simulink library "Lib_Piccolo"  (R2018b)
settings: Solver=VariableStepAuto  StartTime=0.0  StopTime=10.0  RelTol=1e-3
values from neighbouring files (symbols this model uses):
  AccelErrInt2Brakes = 0.15    [SimulationControlConfig16P.m]    (also in SimulationControlConfig16P_LEGACY.m; SimulationControlConfigTAILLESS.m = 0.2; SimulationControlConfigUTAIL.m = 0.2)
  AileronMax = 25    [SimulationControlConfig16P.m]    (also in SimulationControlConfig16P_LEGACY.m; SimulationControlConfigTAILLESS.m; SimulationControlConfigUTAIL.m)
  AileronPower = 0.00268    [SimulationControlConfig16P.m]    (also in SimulationControlConfig16P_LEGACY.m; SimulationControlConfigTAILLESS.m; SimulationControlConfigUTAIL.m)
  AileronSurfaceMax = 45    [SimulationControlConfig16P.m]    (also in SimulationControlConfig16P_LEGACY.m)
  AileronTrim = 0    [SimulationControlConfig16P.m]    (also in SimulationControlConfig16P_LEGACY.m; SimulationControlConfigTAILLESS.m; SimulationControlConfigUTAIL.m)
  Alt = 1000 + TerrainHeight    [SimulationStateConfig.m]
  AltCruise_m = testPlans(testIndx).terrainElevation * 0.3048 + 200    [SimulationControlConfig16P.m]    (also in SimulationControlConfigTAILLESS.m = 1083; SimulationControlConfigUTAIL.m = testPlans(testIndx).terrainElevation * 0.3048 + 152)
  AltitudeRate2PitchCmdIntegratorInit = 0.1    [SimulationControlPre.m]
  AltMax = 10000    [SimulationControlConfig16P.m]    (also in SimulationControlConfig16P_LEGACY.m; SimulationControlConfigTAILLESS.m; SimulationControlConfigUTAIL.m)
  AltMaxAccel = 1.25    [SimulationControlConfig16P.m]    (also in SimulationControlConfig16P_LEGACY.m = 0.9; SimulationControlConfigTAILLESS.m = 1.7; SimulationControlConfigUTAIL.m = 2)
  AltMin = 0    [SimulationControlConfig16P.m]    (also in SimulationControlConfig16P_LEGACY.m; SimulationControlConfigTAILLESS.m; SimulationControlConfigUTAIL.m)
  AltRateCmd2Pitch = 0.50    (= 0.5)    [SimulationControlConfig16P.m]    (also in SimulationControlConfig16P_LEGACY.m = 0.6; SimulationControlConfigTAILLESS.m = 0.2; SimulationControlConfigUTAIL.m = 0.3)
  AltRateError2Pitch = 0.40    (= 0.4)    [SimulationControlConfig16P.m]    (also in SimulationControlConfig16P_LEGACY.m; SimulationControlConfigTAILLESS.m = 0.55; SimulationControlConfigUTAIL.m = 0.55)
  AltRateErrorInt2Pitch = 0.50    (= 0.5)    [SimulationControlConfig16P.m]    (also in SimulationControlConfig16P_LEGACY.m = 0.45; SimulationControlConfigTAILLESS.m; SimulationControlConfigUTAIL.m = 0.75)
  AltRateLpfCutOff = 3    [SimulationControlConfig16P.m]    (also in SimulationControlConfig16P_LEGACY.m; SimulationControlConfigTAILLESS.m = 2; SimulationControlConfigUTAIL.m = 2)
  AutoNosegear2Rudder = 26    [SimulationControlConfig16P.m]    (also in SimulationControlConfig16P_LEGACY.m; SimulationControlConfigTAILLESS.m = 25.2; SimulationControlConfigUTAIL.m = 14)
  b = 5.54    [SimulationControlConfig16P.m]    (also in SimulationControlConfig16P_LEGACY.m; SimulationControlConfigTAILLESS.m = 2.37; SimulationControlConfigUTAIL.m = 2.37)
  Bank2AileronIntegratorInit = 0    [SimulationControlPre.m]
  BankMax_User = BankMax_User/180*pi    (= 0.523598775598)    [SimulationControlConfig16P.m]    (also in SimulationControlConfig16P_LEGACY.m; SimulationControlConfigTAILLESS.m = 0.610865238198; SimulationControlConfigUTAIL.m = 0.628318530718)
  baseLegFlaps = 20    [SimulationControlConfig16P.m]    (also in SimulationControlConfig16P_LEGACY.m = 0; SimulationControlConfigTAILLESS.m = 15; SimulationControlConfigUTAIL.m = 10)
  C = GeneticOpt.C    [SimulationCostFunction.m]
  c = Sw/b    (= 0.841696750903)    [SimulationControlConfig16P.m]    (also in SimulationControlConfig16P_LEGACY.m; SimulationControlConfigTAILLESS.m = 0.354008438819; SimulationControlConfigUTAIL.m = 0.354008438819)
  cell2WheelFactorMG = 5.98    [SimulationSensorConfig16P_LEGACY.m]
  cell2WheelFactorNG = 1    [SimulationSensorConfig16P_LEGACY.m]
  cellSatMaxMG = 15000    [SimulationSensorConfig16P.m]    (also in SimulationSensorConfig16P_LEGACY.m; SimulationSensorConfigTAILLESS7P.m; SimulationSensorConfigUTAIL7P.m)
  cellSatMaxNG = 1000    [SimulationSensorConfig16P.m]    (also in SimulationSensorConfig16P_LEGACY.m; SimulationSensorConfigTAILLESS7P.m; SimulationSensorConfigUTAIL7P.m)
  cellSatMinMG = -15000    [SimulationSensorConfig16P.m]    (also in SimulationSensorConfig16P_LEGACY.m; SimulationSensorConfigTAILLESS7P.m; SimulationSensorConfigUTAIL7P.m)
  cellSatMinNG = -1000    [SimulationSensorConfig16P.m]    (also in SimulationSensorConfig16P_LEGACY.m; SimulationSensorConfigTAILLESS7P.m; SimulationSensorConfigUTAIL7P.m)
  CL_Limit = CL_Max    (= 0.54)    [SimulationControlConfig16P.m]    (also in SimulationControlConfig16P_LEGACY.m; SimulationControlConfigTAILLESS.m; SimulationControlConfigUTAIL.m = 0.53)
  CL_Max = 0.54    [SimulationControlConfig16P.m]    (also in SimulationControlConfig16P_LEGACY.m; SimulationControlConfigTAILLESS.m; SimulationControlConfigUTAIL.m = 0.53)
  CL_Max_Nom = 0.465    [SimulationControlConfig16P.m]    (also in SimulationControlConfig16P_LEGACY.m; SimulationControlConfigTAILLESS.m = 0.39; SimulationControlConfigUTAIL.m)
  CL_Min = 0    [SimulationControlConfig16P.m]    (also in SimulationControlConfig16P_LEGACY.m; SimulationControlConfigTAILLESS.m; SimulationControlConfigUTAIL.m)
  ClimbMaxFraction = 0.35    [SimulationControlConfig16P.m]    (also in SimulationControlConfig16P_LEGACY.m = 0.24; SimulationControlConfigTAILLESS.m = 0.19; SimulationControlConfigUTAIL.m = 0.21)
  ClimboutMaxBank = 7.0    (= 7)    [SimulationControlConfig16P.m]    (also in SimulationControlConfig16P_LEGACY.m; SimulationControlConfigTAILLESS.m = 5; SimulationControlConfigUTAIL.m)
  ClimboutTimer = 7.0    (= 7)    [SimulationControlConfig16P.m]    (also in SimulationControlConfig16P_LEGACY.m; SimulationControlConfigTAILLESS.m; SimulationControlConfigUTAIL.m)
  dCl_per_dFlap = 0.005581818    [SimulationControlConfig16P.m]    (also in SimulationControlConfig16P_LEGACY.m = 0; SimulationControlConfigTAILLESS.m = 0; SimulationControlConfigUTAIL.m = 0)
  DecelerationCmd = 3.1    [SimulationControlConfig16P.m]    (also in SimulationControlConfig16P_LEGACY.m; SimulationControlConfigTAILLESS.m = 0.1; SimulationControlConfigUTAIL.m = 0.1)
  DeRotateLogicEndTimer = abs((NoseDownLimit_Deg-1)/DeRotateRamp_Dps)    [SimulationControlConfig16P.m]    (also in SimulationControlConfig16P_LEGACY.m; SimulationControlConfigTAILLESS.m; SimulationControlConfigUTAIL.m)
  DeRotateLogicHoldNoseUpTimer = 0.1    [SimulationControlConfig16P.m]    (also in SimulationControlConfig16P_LEGACY.m; SimulationControlConfigTAILLESS.m; SimulationControlConfigUTAIL.m)
  DeRotateLogicTimerTimeout = 2    [SimulationControlConfig16P.m]    (also in SimulationControlConfig16P_LEGACY.m; SimulationControlConfigTAILLESS.m; SimulationControlConfigUTAIL.m)
  DeRotateLowerCmdSaturation = 0    [SimulationControlConfig16P.m]    (also in SimulationControlConfig16P_LEGACY.m; SimulationControlConfigTAILLESS.m; SimulationControlConfigUTAIL.m)
  DeRotateRamp_Dps = 3    [SimulationControlConfig16P.m]    (also in SimulationControlConfig16P_LEGACY.m; SimulationControlConfigTAILLESS.m = 8; SimulationControlConfigUTAIL.m = 8)
  DeRotateUpperCmdSaturation = 7    [SimulationControlConfig16P.m]    (also in SimulationControlConfig16P_LEGACY.m; SimulationControlConfigTAILLESS.m; SimulationControlConfigUTAIL.m)
  DescentMaxFraction = 0.22    [SimulationControlConfig16P.m]    (also in SimulationControlConfig16P_LEGACY.m = 0.2; SimulationControlConfigTAILLESS.m = 0.17; SimulationControlConfigUTAIL.m = 0.17)
  DesktopSimTerrainOffset_m = 0.406    [SimulationAircraftConfig.m]
  downwindFlaps = 0    [SimulationControlConfig16P.m]    (also in SimulationControlConfig16P_LEGACY.m; SimulationControlConfigTAILLESS.m; SimulationControlConfigUTAIL.m)
  DP_init = 0.5*1.225*V_init^2    [SimulationControlConfig16P.m]    (also in SimulationControlConfig16P_LEGACY.m; SimulationControlConfigTAILLESS.m; SimulationControlConfigUTAIL.m)
  dscNoiseMG = 1    [SimulationSensorConfig16P_LEGACY.m]
  dscNoiseNG = 0.25    [SimulationSensorConfig16P_LEGACY.m]
  DSCnumBits = 24    [SimulationSensorConfig16P.m]    (also in SimulationSensorConfig16P_LEGACY.m; SimulationSensorConfigTAILLESS7P.m; SimulationSensorConfigUTAIL7P.m)
  DSCRangeMaxMG = 15000    [SimulationSensorConfig16P.m]    (also in SimulationSensorConfig16P_LEGACY.m; SimulationSensorConfigTAILLESS7P.m; SimulationSensorConfigUTAIL7P.m)
  DSCRangeMaxNG = 1000    [SimulationSensorConfig16P.m]    (also in SimulationSensorConfig16P_LEGACY.m; SimulationSensorConfigTAILLESS7P.m; SimulationSensorConfigUTAIL7P.m)
  DSCRangeMinMG = -15000    [SimulationSensorConfig16P.m]    (also in SimulationSensorConfig16P_LEGACY.m; SimulationSensorConfigTAILLESS7P.m; SimulationSensorConfigUTAIL7P.m)
  DSCRangeMinNG = -1000    [SimulationSensorConfig16P.m]    (also in SimulationSensorConfig16P_LEGACY.m; SimulationSensorConfigTAILLESS7P.m; SimulationSensorConfigUTAIL7P.m)
  dt = DLLSim.dt    [SimulationTimeStep.m]    (also in SimulationTrim.m = 0.02)
  EarlyTouchdownThreshold = 3.0    (= 3)    [SimulationControlConfig16P.m]    (also in SimulationControlConfig16P_LEGACY.m; SimulationControlConfigTAILLESS.m = 2.2; SimulationControlConfigUTAIL.m = 2.5)
  ElevatorDeflectionRate = 15    [SimulationControlConfig16P.m]    (also in SimulationControlConfig16P_LEGACY.m = 12; SimulationControlConfigTAILLESS.m = 10; SimulationControlConfigUTAIL.m = 12)
  ElevatorMax = 25    [SimulationControlConfig16P.m]    (also in SimulationControlConfig16P_LEGACY.m; SimulationControlConfigTAILLESS.m; SimulationControlConfigUTAIL.m)
  ElevatorPower = -0.002209    [SimulationControlConfig16P.m]    (also in SimulationControlConfig16P_LEGACY.m; SimulationControlConfigTAILLESS.m = -0.002956; SimulationControlConfigUTAIL.m = -0.00205983)
  ElevatorTrim = -3.5    [SimulationControlConfig16P.m]    (also in SimulationControlConfig16P_LEGACY.m; SimulationControlConfigTAILLESS.m = -6; SimulationControlConfigUTAIL.m = -8)
  elevonBias = 0    [SimulationControlConfig16P.m]    (also in SimulationControlConfig16P_LEGACY.m; SimulationControlConfigTAILLESS.m; SimulationControlConfigUTAIL.m)
  Enable_TAS_Protection = 0    [SimulationControlConfig16P.m]    (also in SimulationControlConfig16P_LEGACY.m; SimulationControlConfigTAILLESS.m; SimulationControlConfigUTAIL.m)
  EnableCrossTrackAbort = 1    [SimulationControlConfig16P.m]    (also in SimulationControlConfigTAILLESS.m; SimulationControlConfigUTAIL.m)
  EnergyBandwidth = 0.02    [SimulationControlConfig16P.m]    (also in SimulationControlConfig16P_LEGACY.m; SimulationControlConfigTAILLESS.m = 0.06; SimulationControlConfigUTAIL.m = 0.06)
  EngineLhFuelCut = 0    [SimulationAircraftConfig.m]
  EngineRhFuelCut = 0    [SimulationAircraftConfig.m]
  FastThrottleRate = 0.075    [SimulationControlConfig16P.m]    (also in SimulationControlConfig16P_LEGACY.m = 0.05; SimulationControlConfigTAILLESS.m = 0.1; SimulationControlConfigUTAIL.m = 0.1)
  FilterWarmUpTime = 2    [SimulationSensorConfig16P.m]    (also in SimulationSensorConfig16P_LEGACY.m; SimulationSensorConfigTAILLESS7P.m; SimulationSensorConfigUTAIL7P.m)
  finalApproachFlaps = 20    [SimulationControlConfig16P.m]    (also in SimulationControlConfig16P_LEGACY.m = 0; SimulationControlConfigTAILLESS.m = 22; SimulationControlConfigUTAIL.m = 10)
  FinalDescentSlope_Deg = testPlans(testIndx).descentSlope    [SimulationControlConfig16P.m]    (also in SimulationControlConfig16P_LEGACY.m; SimulationControlConfigTAILLESS.m; SimulationControlConfigUTAIL.m)
  flapMax = 0    [SimulationControlConfig16P.m]    (also in SimulationControlConfig16P_LEGACY.m; SimulationControlConfigTAILLESS.m; SimulationControlConfigUTAIL.m)
  flapRate = 7.5    [SimulationControlConfig16P.m]    (also in SimulationControlConfig16P_LEGACY.m; SimulationControlConfigTAILLESS.m = 6.6; SimulationControlConfigUTAIL.m)
  FlareHeight = 5    [SimulationControlConfig16P.m]    (also in SimulationControlConfig16P_LEGACY.m = 4.8; SimulationControlConfigTAILLESS.m = 2.5; SimulationControlConfigUTAIL.m = 2)
  FlareVerticalRate_mps = -0.4    [SimulationControlConfig16P.m]    (also in SimulationControlConfig16P_LEGACY.m = -0.5; SimulationControlConfigTAILLESS.m = -0.15; SimulationControlConfigUTAIL.m = -0.15)
  Fp_Aileron = 0.55*2*pi*RollRateLpfCutoff*dt    [SimulationControlConfig16P.m]    (also in SimulationControlConfig16P_LEGACY.m; SimulationControlConfigTAILLESS.m; SimulationControlConfigUTAIL.m)
  Fp_Alt = 0.55*AltBandwidth    (= 0.099)    [SimulationControlConfig16P.m]    (also in SimulationControlConfig16P_LEGACY.m; SimulationControlConfigTAILLESS.m = 0.587477826221; SimulationControlConfigUTAIL.m = 0.69115038379)
  Fp_AltRate = 0.55*2*pi*AltRateLpfCutOff*dt    [SimulationControlConfig16P.m]    (also in SimulationControlConfig16P_LEGACY.m; SimulationControlConfigTAILLESS.m; SimulationControlConfigUTAIL.m)
  Fp_Elevator = 0.55*2*pi*PitchRateLpfCutoff*dt    [SimulationControlConfig16P.m]    (also in SimulationControlConfig16P_LEGACY.m; SimulationControlConfigTAILLESS.m; SimulationControlConfigUTAIL.m)
  Fp_Energy = 0.55*2*pi*EnergyBandwidth    (= 0.069115038379)    [SimulationControlConfig16P.m]    (also in SimulationControlConfig16P_LEGACY.m; SimulationControlConfigTAILLESS.m = 0.207345115137; SimulationControlConfigUTAIL.m = 0.207345115137)
  Fp_Energy2 = 0.55*2*pi*EnergyBandwidth*dt    [SimulationControlConfig16P.m]    (also in SimulationControlConfig16P_LEGACY.m; SimulationControlConfigTAILLESS.m; SimulationControlConfigUTAIL.m)
  Fp_Pitch = 0.55*2*pi*PitchBandwidth    (= 2.76460153516)    [SimulationControlConfig16P.m]    (also in SimulationControlConfig16P_LEGACY.m = 3.11017672705; SimulationControlConfigTAILLESS.m = 3.80132711084; SimulationControlConfigUTAIL.m = 2.41902634326)
  Fp_Pitch_2 = 0.55*2*pi*PitchBandwidth*dt    [SimulationControlConfig16P.m]    (also in SimulationControlConfig16P_LEGACY.m; SimulationControlConfigTAILLESS.m; SimulationControlConfigUTAIL.m)
  Fp_Roll = RollBandwidth^2    (= 1)    [SimulationControlConfig16P.m]    (also in SimulationControlConfig16P_LEGACY.m = 1.44; SimulationControlConfigTAILLESS.m; SimulationControlConfigUTAIL.m)
  Fp_Rudder = 0.55*2*pi*YawRateLpfCutoff*dt    [SimulationControlConfig16P.m]    (also in SimulationControlConfig16P_LEGACY.m; SimulationControlConfigTAILLESS.m; SimulationControlConfigUTAIL.m)
  Fp_TAS = 0.55*2*pi*TASBandwidth    (= 0.103672557568)    [SimulationControlConfig16P.m]    (also in SimulationControlConfig16P_LEGACY.m; SimulationControlConfigTAILLESS.m = 0.172787595947; SimulationControlConfigUTAIL.m = 0.172787595947)
  Fp_TAS_Filter = 2*pi*TasLpfCutoff*dt    [SimulationControlConfig16P.m]    (also in SimulationControlConfig16P_LEGACY.m; SimulationControlConfigTAILLESS.m; SimulationControlConfigUTAIL.m)
  Fp_Turn = 0.55*2*pi*TurnErrLPFcutoff    (= 0.0345575191895)    [SimulationControlConfig16P.m]    (also in SimulationControlConfig16P_LEGACY.m; SimulationControlConfigTAILLESS.m = 0.172787595947; SimulationControlConfigUTAIL.m = 0.172787595947)
  Fp_TurnDerr = 0.55*2*pi*TurnDerivativeLPFcutoff    (= 0.0345575191895)    [SimulationControlConfig16P.m]    (also in SimulationControlConfig16P_LEGACY.m; SimulationControlConfigTAILLESS.m = 0.172787595947; SimulationControlConfigUTAIL.m = 0.172787595947)
  FTV = 3    [SimulationAircraftConfig.m]
  ftvStaticPositionError = 1/1.18    (= 0.847457627119)    [SimulationSensorConfig16P.m]    (also in SimulationSensorConfig16P_LEGACY.m; SimulationSensorConfigTAILLESS7P.m = 1; SimulationSensorConfigUTAIL7P.m = 1)
  g = 9.81    [SimulationStateConfig.m]
  GustSpd_Kts = testPlans(testIndx).gustSpd    [SimulationStateConfig.m]
  GustTriggerVal = testPlans(testIndx).gustTriggerVal    [SimulationStateConfig.m]
  HeadingErr2TurnRate = 0.5    [SimulationControlConfig16P.m]    (also in SimulationControlConfig16P_LEGACY.m; SimulationControlConfigTAILLESS.m; SimulationControlConfigUTAIL.m)
  HeadingErrDer2TurnRate = 0.3    [SimulationControlConfig16P.m]    (also in SimulationControlConfig16P_LEGACY.m; SimulationControlConfigTAILLESS.m; SimulationControlConfigUTAIL.m)
  IASbounce = IASstall*0.8    [SimulationControlPre.m]
  IAScruiseCMD = sqrt(2*m*9.81/(1.225*Sw*CL_cruise))    [SimulationControlConfig16P.m]    (also in SimulationControlConfig16P_LEGACY.m; SimulationControlConfigTAILLESS.m; SimulationControlConfigUTAIL.m)
  IASfinalCMD = 1.12 * IASmin    [SimulationControlConfig16P.m]    (also in SimulationControlConfig16P_LEGACY.m = 1.10 * IASmin; SimulationControlConfigTAILLESS.m = 1.10 * IASmin; SimulationControlConfigUTAIL.m = 1.15 * IASmin)
  IASflareCMD = IASstall    [SimulationControlConfig16P.m]    (also in SimulationControlConfig16P_LEGACY.m; SimulationControlConfigTAILLESS.m; SimulationControlConfigUTAIL.m)
  IASmax = 64    [SimulationControlConfig16P.m]    (also in SimulationControlConfig16P_LEGACY.m = 46; SimulationControlConfigTAILLESS.m = 38.58; SimulationControlConfigUTAIL.m = 35)
  IASmin = sqrt(2*m*9.81/(1.225*Sw*0.9*CL_Max_Nom))    [SimulationControlConfig16P.m]    (also in SimulationControlConfig16P_LEGACY.m; SimulationControlConfigTAILLESS.m; SimulationControlConfigUTAIL.m)
  IASshortCMD = IASstall    [SimulationControlConfig16P.m]    (also in SimulationControlConfig16P_LEGACY.m; SimulationControlConfigTAILLESS.m; SimulationControlConfigUTAIL.m)
  IASstall = sqrt(2*m*9.81/(1.225*Sw*CL_Max))    [SimulationControlConfig16P.m]    (also in SimulationControlConfig16P_LEGACY.m; SimulationControlConfigTAILLESS.m; SimulationControlConfigUTAIL.m)
  inFlight = 1    [SimulationControlConfig16P.m]    (also in SimulationControlConfigTAILLESS.m; SimulationControlConfigUTAIL.m)
  JetCatOffset = 5    [SimulationControlConfig16P.m]    (also in SimulationControlConfig16P_LEGACY.m)
  LaunchRollingElevator = -1.5    [SimulationControlConfig16P.m]    (also in SimulationControlConfig16P_LEGACY.m; SimulationControlConfigTAILLESS.m = 1; SimulationControlConfigUTAIL.m = 1)
  ldg_NosegearMax = 10    [SimulationControlConfig16P.m]    (also in SimulationControlConfig16P_LEGACY.m; SimulationControlConfigTAILLESS.m; SimulationControlConfigUTAIL.m)
  ldg_TrackVyErrInt2Nosegear = 0.1250    (= 0.125)    [SimulationControlConfig16P.m]    (also in SimulationControlConfig16P_LEGACY.m; SimulationControlConfigTAILLESS.m = 0.00714285714286; SimulationControlConfigUTAIL.m = 0.00714285714286)
  ldg_TrackVyErrPro2Nosegear = 0.35    [SimulationControlConfig16P.m]    (also in SimulationControlConfig16P_LEGACY.m; SimulationControlConfigTAILLESS.m = 0.0546666666667; SimulationControlConfigUTAIL.m = 0.0546666666667)
  ldg_TrackY2Vy = 0.07    [SimulationControlConfig16P.m]    (also in SimulationControlConfig16P_LEGACY.m; SimulationControlConfigTAILLESS.m = 0.17; SimulationControlConfigUTAIL.m = 0.17)
  ldg_Vy2NosegearScalingPower = 1.075    [SimulationControlConfig16P.m]    (also in SimulationControlConfig16P_LEGACY.m; SimulationControlConfigTAILLESS.m = 0.6; SimulationControlConfigUTAIL.m = 0.5)
  ldg_Y2VyScalingPower = 0.175    [SimulationControlConfig16P.m]    (also in SimulationControlConfig16P_LEGACY.m; SimulationControlConfigTAILLESS.m = 0; SimulationControlConfigUTAIL.m = 0)
  ldg_YawRate2Nosegear = 0.175    [SimulationControlConfig16P.m]    (also in SimulationControlConfig16P_LEGACY.m; SimulationControlConfigTAILLESS.m = 0.065; SimulationControlConfigUTAIL.m = 0.065)
  LiftSlope = 0.064285    [SimulationControlConfig16P.m]    (also in SimulationControlConfig16P_LEGACY.m; SimulationControlConfigTAILLESS.m = 0.058631; SimulationControlConfigUTAIL.m)
  LPFaileronInit = 0    [SimulationControlPre.m]
  LPFclestInit = 0    [SimulationControlPre.m]
  LPFenergyFFInit = 0    [SimulationControlPre.m]
  LPFtasInit = V_init + 2    [SimulationControlPre.m]
  LPFthrottleInit = ThrottleTrim    [SimulationControlPre.m]
  LPFturnErrInit = 0    [SimulationControlPre.m]
  ... (+115 more)
undefined symbols (not defined in the file or in its folder): abortFlag, alphaHPF, apmDelay, BRWNOUT, CRAWOR, CRAWUR, DiscIntNeverNeededParam, DLLSim, DLLSimStep, ECOMOR, ECOMUR, Fp_Tas, GustTrigger_HeightAgl_m, IPSTAT, LCINTEG, Ldg_Persist_Time, LOWER_FLAGS, MSG_ENABLE, NoiseStd, OLDVAL, OVERRIDE_ENABLE, OVERRIDE_VALUE, REBOOT, reversionEnable, revIASMax, revIASMin, revPitchMax, revPitchMin, revPitchRateMax, revRollMax, revRollRateMax, SAMPLE, SCALON, SensorModel, sigbuilder_block, Sim_Vx, Sim_Vy, Sim_Vz, Sim_Xpos, Sim_Ypos, Sim_Zpos, SYSOR, SYSUR, TARE, TEMPOR, TEMPUR, testIndx, testPlan, testPlans, Trim_piccoloInCmd, Trim_REFSI_FD_IN_nmodeCgShifterCmd_Ft, Trim_REFSI_FD_IN_nmodeFlapLhIBCmd_Deg, Trim_REFSI_FD_IN_nmodeFlapLhOBCmd_Deg, Trim_REFSI_FD_IN_nmodeFlapRhIBCmd_Deg, Trim_REFSI_FD_IN_nmodeFlapRhOBCmd_Deg, Trim_REFSI_FD_IN_nmodeSlatLhCmd_Deg, Trim_REFSI_FD_IN_nmodeSlatRhCmd_Deg, Trim_REFSI_FD_IN_nmodeSplrLhInbdCmd_Deg, Trim_REFSI_FD_IN_nmodeSplrLhOutbdCmd_Deg ... (+5)
libraries: simulink x866, aerolibconvert2 x60, $bdroot x52, aerolibatmos2 x5, dspswit3 x5, simulink_extras x4, dsparch4 x2, Lib_Piccolo_Alt x2, eeGeneralControl x1, dspindex x1
(part 9 of 44)

== system Lib_Piccolo/Altitude Rate to Pitch Command/LPF Vrate2PitchCmd ==
  Input : Inport
  Reset : Inport  Port=2
  ResetValue : Inport  Port=3
  Add1 : Sum  Inputs=++|
  Compare To Constant2 : simulink/Logic and Bit Operations/Compare To Constant  relop=>  const=0  OutDataTypeStr=uint8
  Constant11 : Constant  Value=AltRateLpfCutOff
  Switch : Switch  Criteria=u2 > Threshold
  Switch1 : Switch  Criteria=u2 > Threshold
  Unit Delay1 : UnitDelay  InitialCondition=LPFvRate2PitchInit*pi/180  SampleTime=-1
  a1 : Gain  Gain=1-Fp_AltRate
  b0 : Gain  Gain=Fp_AltRate
  Output : Outport
  wires:
  Constant11/1 -> Compare To Constant2/1
  Compare To Constant2/1 -> Switch1/2
  Switch1/1 -> Output/1
  a1/1 -> Add1/1
  Unit Delay1/1 -> a1/1
  b0/1 -> Add1/2
  Add1/1 -> Switch/3, Switch1/1
  Input/1 -> b0/1, Switch1/3
  Switch/1 -> Unit Delay1/1
  Reset/1 -> Switch/2
  ResetValue/1 -> Switch/1

== system Lib_Piccolo/Altitude Rate to Pitch Command/Latch ==
  D : Inport
  Enable/!Rst : Inport  Port=2
  AND : Logic  IconShape=distinctive  AllPortsSameDT=off  OutDataTypeStr=boolean
  Constant : Constant
  OR : Logic  Operator=OR  IconShape=distinctive  AllPortsSameDT=off  OutDataTypeStr=boolean
  Switch : Switch  Criteria=u2 > Threshold  Threshold=0.5
  Unit Delay : UnitDelay  SampleTime=-1
  Q_Latched : Outport
  wires:
  Unit Delay/1 -> OR/2
  Switch/1 -> Q_Latched/1, Unit Delay/1
  D/1 -> Switch/3, OR/1
  OR/1 -> AND/1
  AND/1 -> Switch/2
  Enable/!Rst/1 -> AND/2
  Constant/1 -> Switch/1

== system Lib_Piccolo/Altitude Rate to Pitch Command/Optimisation Cost ==
  Sim.VRate Error : Inport
  PitchCmd : Inport  Port=2
  Bus Creator : BusCreator  Inputs=4
  Constant : Constant  Value=0
  Constant1 : Constant
  Discrete Derivative : simulink/Discrete/Discrete Derivative  gainval=1.0  ICPrevScaledInput=0.0  OutMin=[]  OutMax=[]  OutDataType=fixdt(1, 16)  OutScaling=2^-10  DoSatur=off
  Display{,1..2,8} (4 alike) : Display
  Gain2 : Gain  Gain=Q
  Gain3 : Gain  Gain=R
  Gain4 : Gain  Gain=C
  Integrator2 : Integrator
  Integrator3 : Integrator
  Integrator7 : Integrator
  Minus : Sum  Inputs=+-
  Multiply3 : Product
  Multiply4 : Product
  Multiply5 : Product
  Pitch Trim : Constant  Value=4
  Rad2Deg : Gain  Gain=180/pi
  Square : Math  Operator=square  SaturateOnIntegerOverflow=on
  Square1 : Math  Operator=square  SaturateOnIntegerOverflow=on
  Square2 : Math  Operator=square  SaturateOnIntegerOverflow=on
  Sum4 : Sum  Inputs=|+++
  Switch : Switch  Criteria=u2 > Threshold
  To Workspace : ToWorkspace  VariableName=COST  SaveFormat=Timeseries  SampleTime=-1
  To Workspace1 : ToWorkspace  VariableName=COST_ALL  SaveFormat=Timeseries  SampleTime=-1
  wires:
  Multiply4/1 -> Integrator2/1
  Integrator2/1 -> Sum4/1, Display1/1, Bus Creator/2  "COST_AltRateError"
  Sum4/1 -> Display/1, Bus Creator/1, To Workspace/1  "COST"
  Switch/1 -> Multiply3/1, Multiply5/1, Multiply4/1
  Discrete Derivative/1 -> Square2/1
  Integrator7/1 -> Display8/1, Bus Creator/4, Sum4/3  "COST_PitchCmdRate"
  Gain3/1 -> Multiply5/2  "Cost_Command"
  Square1/1 -> Gain3/1
  Bus Creator/1 -> To Workspace1/1
  Gain2/1 -> Multiply4/2  "Cost_AltRateError"
  Multiply5/1 -> Integrator3/1
  Sim.VRate Error/1 -> Square/1
  Gain4/1 -> Multiply3/2  "Cost_CommRate"
  Rad2Deg/1 -> Discrete Derivative/1, Minus/1
  Square2/1 -> Gain4/1
  Pitch Trim/1 -> Minus/2
  Square/1 -> Gain2/1
  Constant1/1 -> Switch/3
  [FlareFlag] -> Switch/2
  Constant/1 -> Switch/1
  Multiply3/1 -> Integrator7/1
  Integrator3/1 -> Bus Creator/3, Display2/1, Sum4/2  "COST_PitchCmdMag"
  Minus/1 -> Square1/1
  PitchCmd/1 -> Rad2Deg/1

== system Lib_Piccolo/Altitude Rate to Pitch Command/TASLimit ==
  note: TAS saturates at ~ 100mps which in IAS is 6125Pa
  <V_mps> : Inport
  Saturation Dynamic1 : simulink/Discontinuities/Saturation Dynamic  OutMin=[]  OutMax=[]  OutDataTypeStr=Inherit: Same as second input  OutDataType=fixdt(1, 16)  OutScaling=2^-10  DoSatur=off
  TASmax : Constant  Value=100
  TASmin : Constant  Value=5
  V_mps_Limit : Outport
  wires:
  TASmin/1 -> Saturation Dynamic1/3
  TASmax/1 -> Saturation Dynamic1/1
  <V_mps>/1 -> Saturation Dynamic1/2
  Saturation Dynamic1/1 -> V_mps_Limit/1

== system Lib_Piccolo/Altitude Rate to Pitch Command/Triggered Subsystem ==
  In1 : Inport
  Trigger : TriggerPort  TriggerType=falling  VariantControl=Variant
  Out1 : Outport
  wires:
  In1/1 -> Out1/1

== system Lib_Piccolo/Altitude Rate to Pitch Command LEGACY DEROTATE/DeRotate Logic rev 2 ==
  PitchAngle_Deg : Inport
  Pic_ApMode : Inport  Port=2
  Pic_GlobalOn : Inport  Port=3
  Pic_AssistMode : Inport  Port=4
  WoWBool : Inport  Port=5
  AND : Logic  IconShape=distinctive  AllPortsSameDT=off  OutDataTypeStr=boolean
  AND1 : Logic  IconShape=distinctive  AllPortsSameDT=off  OutDataTypeStr=boolean
  AND2 : Logic  IconShape=distinctive  AllPortsSameDT=off  OutDataTypeStr=boolean
  Compare To Constant1 : simulink/Logic and Bit Operations/Compare To Constant  relop===  const=1  OutDataTypeStr=uint8
  Compare To Constant2 : simulink/Logic and Bit Operations/Compare To Constant  relop===  const=0  OutDataTypeStr=uint8
  Compare To Constant3 : simulink/Logic and Bit Operations/Compare To Constant  relop=<=  const=NoseDownLimit_Deg  OutDataTypeStr=uint8
  Compare To Constant4 : simulink/Logic and Bit Operations/Compare To Constant  relop===  const=10  OutDataTypeStr=uint8
  Compare To Constant5 : simulink/Logic and Bit Operations/Compare To Constant  relop===  const=9  OutDataTypeStr=uint8
  Compare To Constant6 : simulink/Logic and Bit Operations/Compare To Constant  relop===  const=0  OutDataTypeStr=uint8
  Compare To Constant7 : simulink/Logic and Bit Operations/Compare To Constant  relop===  const=11  OutDataTypeStr=uint8
  Constant : Constant  Value=0
  Constant4 : Constant  Value=0
  Constant5 : Constant  Value=-1*DeRotateRamp_Dps
  Data Type Conversion{1..4} (4 alike) : DataTypeConversion
  Discrete-Time Integrator : DiscreteIntegrator  ExternalReset=level  InitialConditionSource=external  SampleTime=-1  LimitOutput=on  UpperSaturationLimit=DeRotateUpperCmdSaturation  LowerSaturationLimit=DeRotateLowerCmdSaturation  ICPrevOutput=DiscIntNeverNeededParam  ICPrevScaledInput=DiscIntNeverNeededParam
  Latch : Subsystem
  Multiply : Product
  Multiply1 : Product  Inputs=3
  NOT : Logic  Operator=NOT  IconShape=distinctive  AllPortsSameDT=off  OutDataTypeStr=boolean
  NOT1 : Logic  Operator=NOT  IconShape=distinctive  AllPortsSameDT=off  OutDataTypeStr=boolean
  OR : Logic  Operator=OR  IconShape=distinctive  AllPortsSameDT=off  OutDataTypeStr=boolean
  OR1 : Logic  Operator=OR  IconShape=distinctive  AllPortsSameDT=off  OutDataTypeStr=boolean
  Saturation : Saturate  UpperLimit=DeRotateUpperCmdSaturation  LowerLimit=DeRotateLowerCmdSaturation
  Switch1 : Switch  Criteria=u2 ~= 0  Threshold=0.5
  Switch2 : Switch  Threshold=1
  Switch3 : Switch  Threshold=1
  Terminator : Terminator
  Timer : Subsystem  mask{period=DeRotateLogicEndTimer}
      mask prompts: period "Period [s]"
  Timer 2 : Subsystem  mask{period=DeRotateLogicTimerTimeout}
      mask prompts: period "Period [s]"
  Timer1 : Subsystem  mask{period=DeRotateLogicHoldNoseUpTimer}
      mask prompts: period "Period [s]"
  PitchDeRotateCmd : Outport
  DeRotateActive : Outport  Port=2
  WoWBool_Out : Outport  Port=3
  wires:
  AND1/1 -> Data Type Conversion4/1
  AND/1 -> AND1/2
  OR/1 -> AND1/1
  Compare To Constant6/1 -> AND/2
  Compare To Constant1/1 -> AND/1
  Pic_AssistMode/1 -> Compare To Constant6/1
  Pic_GlobalOn/1 -> Compare To Constant1/1
  Multiply/1 -> Timer 2/1(Enable/!Rst), Multiply1/2
  Data Type Conversion2/1 -> Multiply1/3  "DeRotateTimeout"
  NOT/1 -> Data Type Conversion2/1
  Timer 2/1(Expired) -> OR1/1, NOT/1
  PitchAngle_Deg/1 -> Compare To Constant3/1, Saturation/1
  Saturation/1 -> Discrete-Time Integrator/3, Switch3/3
  Multiply1/1 -> Switch1/2, Switch3/2, Timer1/1(Enable/!Rst), Compare To Constant2/1, DeRotateActive/1  "DeRotateActive"
  Switch3/1 -> PitchDeRotateCmd/1  "PitchCmdRotate_Deg"
  Pic_ApMode/1 -> Compare To Constant7/1, Compare To Constant5/1, Compare To Constant4/1
  Switch1/1 -> Terminator/1  "WoWBool_Out"
  Constant4/1 -> Switch1/1
  WoWBool/1 -> AND2/2, Switch1/3, Multiply/2
  Compare To Constant3/1 -> Timer/1(Enable/!Rst)
  Latch/1(Q_Latched) -> NOT1/1, OR1/2
  Data Type Conversion3/1 -> Multiply1/1  "DeRotateCompleteDelayTimer"
  NOT1/1 -> Data Type Conversion3/1
  Compare To Constant4/1 -> OR/1
  Compare To Constant5/1 -> OR/2
  Data Type Conversion4/1 -> Multiply/1
  Discrete-Time Integrator/1 -> Switch3/1  "PitchCmdRotate_Deg"
  Compare To Constant2/1 -> Discrete-Time Integrator/2
  Constant5/1 -> Switch2/1
  Constant/1 -> Switch2/3
  Timer1/1(Expired) -> Data Type Conversion1/1
  Switch2/1 -> Discrete-Time Integrator/1
  Data Type Conversion1/1 -> Switch2/2
  OR1/1 -> AND2/1
  AND2/1 -> WoWBool_Out/1
  Timer/1(Expired) -> Latch/1(D)
  Compare To Constant7/1 -> Latch/2(Enable/!Rst)

== system Lib_Piccolo/Altitude Rate to Pitch Command LEGACY DEROTATE/Integrator ==
  In : Inport
  Reset : Inport  Port=2
  Init : Inport  Port=3
  Enable : EnablePort
  Discrete-Time Integrator : DiscreteIntegrator  ExternalReset=level  InitialConditionSource=external  SampleTime=-1  LimitOutput=on  UpperSaturationLimit=PitchMax  LowerSaturationLimit=-PitchMax  ICPrevOutput=DiscIntNeverNeededParam  ICPrevScaledInput=DiscIntNeverNeededParam
  Out : Outport
  wires:
  In/1 -> Discrete-Time Integrator/1
  Discrete-Time Integrator/1 -> Out/1
  Reset/1 -> Discrete-Time Integrator/2
  Init/1 -> Discrete-Time Integrator/3

== system Lib_Piccolo/Altitude Rate to Pitch Command LEGACY DEROTATE/LPF Vrate2PitchCmd ==
  Input : Inport
  Reset : Inport  Port=2
  Add1 : Sum  Inputs=++|
  Compare To Constant2 : simulink/Logic and Bit Operations/Compare To Constant  relop=>  const=0  OutDataTypeStr=uint8
  Constant11 : Constant  Value=AltRateLpfCutOff
  Switch1 : Switch  Criteria=u2 > Threshold
  Unit Delay1 : UnitDelay  InitialCondition=LPFvRate2PitchInit*pi/180  SampleTime=-1
  a1 : Gain  Gain=1-Fp_AltRate
  b0 : Gain  Gain=Fp_AltRate
  Output : Outport
  wires:
  Constant11/1 -> Compare To Constant2/1
  Compare To Constant2/1 -> Switch1/2
  Switch1/1 -> Output/1
  Input/1 -> b0/1, Switch1/3
  a1/1 -> Add1/1
  Unit Delay1/1 -> a1/1
  b0/1 -> Add1/2
  Add1/1 -> Switch1/1, Unit Delay1/1

== system Lib_Piccolo/Altitude Rate to Pitch Command LEGACY DEROTATE/Latch ==
  D : Inport
  Enable/!Rst : Inport  Port=2
  AND : Logic  IconShape=distinctive  AllPortsSameDT=off  OutDataTypeStr=boolean
  Constant : Constant
  OR : Logic  Operator=OR  IconShape=distinctive  AllPortsSameDT=off  OutDataTypeStr=boolean
  Switch : Switch  Criteria=u2 > Threshold  Threshold=0.5
  Unit Delay : UnitDelay  SampleTime=-1
  Q_Latched : Outport
  wires:
  Unit Delay/1 -> OR/2
  Switch/1 -> Q_Latched/1, Unit Delay/1
  D/1 -> Switch/3, OR/1
  OR/1 -> AND/1
  AND/1 -> Switch/2
  Enable/!Rst/1 -> AND/2
  Constant/1 -> Switch/1

== system Lib_Piccolo/Altitude Rate to Pitch Command LEGACY DEROTATE/Optimisation Cost ==
  Sim.VRate Error : Inport
  PitchCmd : Inport  Port=2
  Bus Creator : BusCreator  Inputs=4
  Constant : Constant  Value=0
  Constant1 : Constant
  Discrete Derivative : simulink/Discrete/Discrete Derivative  gainval=1.0  ICPrevScaledInput=0.0  OutMin=[]  OutMax=[]  OutDataType=fixdt(1, 16)  OutScaling=2^-10  DoSatur=off
  Display{,1..2,8} (4 alike) : Display
  Gain2 : Gain  Gain=Q
  Gain3 : Gain  Gain=R
  Gain4 : Gain  Gain=C
  Integrator2 : Integrator
  Integrator3 : Integrator
  Integrator7 : Integrator
  Minus : Sum  Inputs=+-
  Multiply3 : Product
  Multiply4 : Product
  Multiply5 : Product
  Pitch Trim : Constant  Value=4
  Rad2Deg : Gain  Gain=180/pi
  Square : Math  Operator=square  SaturateOnIntegerOverflow=on
  Square1 : Math  Operator=square  SaturateOnIntegerOverflow=on
  Square2 : Math  Operator=square  SaturateOnIntegerOverflow=on
  Sum4 : Sum  Inputs=|+++
  Switch : Switch  Criteria=u2 > Threshold
  To Workspace : ToWorkspace  VariableName=COST  SaveFormat=Timeseries  SampleTime=-1
  To Workspace1 : ToWorkspace  VariableName=COST_ALL  SaveFormat=Timeseries  SampleTime=-1
  wires:
  Multiply4/1 -> Integrator2/1
  Integrator2/1 -> Sum4/1, Display1/1, Bus Creator/2  "COST_AltRateError"
  Sum4/1 -> Display/1, Bus Creator/1, To Workspace/1  "COST"
  Switch/1 -> Multiply3/1, Multiply5/1, Multiply4/1
  Discrete Derivative/1 -> Square2/1
  Integrator7/1 -> Display8/1, Bus Creator/4, Sum4/3  "COST_PitchCmdRate"
  Gain3/1 -> Multiply5/2  "Cost_Command"
  Square1/1 -> Gain3/1
  Bus Creator/1 -> To Workspace1/1
  Gain2/1 -> Multiply4/2  "Cost_AltRateError"
  Multiply5/1 -> Integrator3/1
  Sim.VRate Error/1 -> Square/1
  Gain4/1 -> Multiply3/2  "Cost_CommRate"
  Rad2Deg/1 -> Discrete Derivative/1, Minus/1
  Square2/1 -> Gain4/1
  Pitch Trim/1 -> Minus/2
  Square/1 -> Gain2/1
  Constant1/1 -> Switch/3
  [FlareFlag] -> Switch/2
  Constant/1 -> Switch/1
  Multiply3/1 -> Integrator7/1
  Integrator3/1 -> Bus Creator/3, Display2/1, Sum4/2  "COST_PitchCmdMag"
  Minus/1 -> Square1/1
  PitchCmd/1 -> Rad2Deg/1

== system Lib_Piccolo/Altitude Rate to Pitch Command LEGACY DEROTATE/Triggered Subsystem ==
  In1 : Inport
  Trigger : TriggerPort  TriggerType=falling  VariantControl=Variant
  Out1 : Outport
  wires:
  In1/1 -> Out1/1

== system Lib_Piccolo/Altitude Reference Model/Alt Max Accel Rate Limit ==
  note: Y(k)
  note: U(k)
  up : Inport
  u : Inport  Port=2
  lo : Inport  Port=3
  Delay Input2 : UnitDelay  Description=Store in Global RAM  DisableCoverage=on  InitialCondition=RateLimitAltAccelInit  SampleTime=-1
  Difference Inputs1 : Sum  Description=Add in CPU  DisableCoverage=on  Inputs=+-  OutDataTypeStr=Inherit: Inherit via back propagation
  Difference Inputs2 : Sum  Description=Add in CPU  OutDataTypeStr=Inherit: Inherit via back propagation
  FixPt Data Type Duplicate : DataTypeDuplicate  DisableCoverage=on  NumInputPorts=7
  Saturation Dynamic2 : simulink/Discontinuities/Saturation Dynamic  OutMin=[]  OutMax=[]  OutDataTypeStr=Inherit: Same as second input  OutDataType=fixdt(1, 16)  OutScaling=2^-10  DoSatur=off
  delta fall limit : Product  DisableCoverage=on  Inputs=**  OutDataTypeStr=Inherit: Inherit via back propagation  SaturateOnIntegerOverflow=on
  delta rise limit : Product  DisableCoverage=on  Inputs=**  OutDataTypeStr=Inherit: Inherit via back propagation  SaturateOnIntegerOverflow=on
  sample time : SampleTimeMath  DisableCoverage=on  TsampMathOp=Ts Only  weightValue=1
  Y : Outport  InitialOutput=0
  wires:
  Difference Inputs2/1 -> Y/1, FixPt Data Type Duplicate/1, Delay Input2/1
  sample time/1 -> delta rise limit/2, delta fall limit/2
  Delay Input2/1 -> FixPt Data Type Duplicate/2, Difference Inputs1/2, Difference Inputs2/2  "Y(k-1)"
  up/1 -> delta rise limit/1
  u/1 -> sample time/1, FixPt Data Type Duplicate/5, Difference Inputs1/1
  Saturation Dynamic2/1 -> FixPt Data Type Duplicate/7, Difference Inputs2/1
  lo/1 -> delta fall limit/1
  delta rise limit/1 -> Saturation Dynamic2/1, FixPt Data Type Duplicate/6
  Difference Inputs1/1 -> Saturation Dynamic2/2, FixPt Data Type Duplicate/4  "( U(k) - Y(k-1) )"
  delta fall limit/1 -> Saturation Dynamic2/3, FixPt Data Type Duplicate/3

== system Lib_Piccolo/Bank to Aileron/Bank Angle Limit Calculation ==
  note: From FWG3 Doc (Page 13) -
      | if (state >= shortFinal)
      | $C_{L-Limit} =C_{L-MAX}$
      | else
      | $C_{L-Limit} = 0.9C_{L-MAX\_NOM}$
      |
      | Adjustments will need to be applied to CL_Limit here,
      | CL_Limit = CL_Limit + dCl/dFlap * dFlap
  note: Leave Aero Load Feature off During Landing Verification
      | (switch in down position)
  apMode : Inport
  Q : Inport  Port=2
  Acos : Trigonometry  Operator=acos
  Compare To Constant1 : simulink/Logic and Bit Operations/Compare To Constant  relop=<=  const=9  OutDataTypeStr=uint8
  Compare To Constant2 : simulink/Logic and Bit Operations/Compare To Constant  relop=>=  const=9  OutDataTypeStr=uint8
  Constant : Constant  Value=Sw
  Constant1 : Constant  Value=CL_Limit
  Constant2 : Constant  Value=m
  Constant3 : Constant  Value=nMax_User
  Constant4 : Constant  Value=nMin_User
  Constant5 : Constant  Value=CL_Min
  Constant6 : Constant
  Constant7 : Constant  Value=0.9*CL_Max_Nom
  Divide : Product  Inputs=*/
  Flap Compensation : $bdroot/Pitch to Elevator/Reference Frame Conversion and Pitch Rate Limit Determination/AeroVsStruct_Limit/Flap Compensation  SystemSampleTime=-1
  Gain9 : Gain  Gain=180/pi
  "Load Factors (nMax,nMin) at current conditions " : MATLAB Function  TreatAsAtomicUnit=on
  Min : MinMax  Inputs=2
  Switch : Switch  Criteria=u2 > Threshold
  Switch1 : Switch  Criteria=u2 > Threshold
  Terminator : Terminator
  Terminator2 : Terminator
  "User and State Machine Limits " : Subsystem
  BankMax_Euler : Outport
  wires:
  Flap Compensation/1 -> "Load Factors (nMax,nMin) at current conditions "/3(CL_Limit)  "Sim.CL_Limit"
  Constant7/1 -> Switch1/3
  Switch1/1 -> Flap Compensation/1
  Constant1/1 -> Switch1/1
  Compare To Constant2/1 -> Switch1/2
  apMode/1 -> "User and State Machine Limits "/1(apMode), Compare To Constant1/1, Compare To Constant2/1
  Switch/1 -> BankMax_Euler/1
  Compare To Constant1/1 -> Switch/2
  "User and State Machine Limits "/1(UserLimit) -> Switch/3, Min/2
  Gain9/1 -> Terminator2/1  "Sim.BanknMax"
  Acos/1 -> Min/1, Gain9/1
  Min/1 -> Switch/1
  Divide/1 -> Acos/1
  Constant6/1 -> Divide/1
  "Load Factors (nMax,nMin) at current conditions "/2(nMin) -> Terminator/1
  Constant5/1 -> "Load Factors (nMax,nMin) at current conditions "/4(CL_Min)
  Constant4/1 -> "Load Factors (nMax,nMin) at current conditions "/7(nMin_User)
  Constant3/1 -> "Load Factors (nMax,nMin) at current conditions "/6(nMax_User)
  Constant2/1 -> "Load Factors (nMax,nMin) at current conditions "/5(m)
  Constant/1 -> "Load Factors (nMax,nMin) at current conditions "/2(Sw)
  "Load Factors (nMax,nMin) at current conditions "/1(nMax) -> Divide/2  "nMax"
  Q/1 -> "Load Factors (nMax,nMin) at current conditions "/1(Q)

== system Lib_Piccolo/Bank to Aileron/Dynamic Inversion PID ==
  RollRateCmd_Euler : Inport
  RollRate_Euler : Inport  Port=2
  Q : Inport  Port=3
  V : Inport  Port=4
  apMode : Inport  Port=5
  1-K_TD : Gain  Gain=1-RollDampingTrust
  1/AileronPower : Gain  Gain=1/AileronPower
  "1/AileronPower  " : Gain  Gain=1/AileronPower
  "AileronTrim " : Constant  Value=AileronTrim
  Compare To Constant1 : simulink/Logic and Bit Operations/Compare To Constant  relop=<=  const=1  OutDataTypeStr=uint8
  Compare To Constant2 : simulink/Logic and Bit Operations/Compare To Constant  relop===  const=11  OutDataTypeStr=uint8
  Constant2 : Constant  Value=Bank2AileronIntegratorInit
  Dimensional Aileron Power : Subsystem
  Discrete-Time Integrator1 : DiscreteIntegrator  IntegratorMethod=Integration: Backward Euler  gainval=1  ExternalReset=level  InitialConditionSource=external  SampleTime=-1  LimitOutput=on  UpperSaturationLimit=AileronMax  LowerSaturationLimit=-AileronMax  ICPrevOutput=DiscIntNeverNeededParam  ICPrevScaledInput=DiscIntNeverNeededParam
  Divide : Product  Inputs=/*
  Gain : Gain  Gain=-1
  Gain1 : Gain
  Gain4 : Gain  Gain=RollRateError2Accel
  KI_Roll : Gain  Gain=RollRateErrorInt2Accel
  K_TD : Gain  Gain=RollDampingTrust
  Kp_Roll : Gain  Gain=RollRateError2Accel
  LPF AileronCmd : Subsystem
  NOT : Logic  Operator=NOT  IconShape=distinctive  AllPortsSameDT=off  OutDataTypeStr=boolean
  NOT1 : Logic  Operator=NOT  IconShape=distinctive  AllPortsSameDT=off  OutDataTypeStr=boolean
  OR : Logic  Operator=OR  IconShape=distinctive  AllPortsSameDT=off  OutDataTypeStr=boolean
  OR1 : Logic  Operator=OR  IconShape=distinctive  AllPortsSameDT=off  OutDataTypeStr=boolean
  Roll Moment Caused By Damping : Subsystem
  Rollout Roll Control : Subsystem
  STIFF : Constant  Value=0
  Saturation : Saturate  UpperLimit=AileronMax  LowerLimit=-AileronMax
  Saturation1 : Saturate  UpperLimit=6125  LowerLimit=200
  Sum : Sum  Inputs=|+-
  Sum1 : Sum  Inputs=|+--+
  Sum2 : Sum  Inputs=|++
  Sum3 : Sum  Inputs=++|
  Switch : Switch  Criteria=u2 > Threshold
  Terminator : Terminator
  Terminator1 : Terminator
  Unit Delay : UnitDelay  SampleTime=-1
  Aileron_Deg : Outport
  wires:
  Saturation1/1 -> Dimensional Aileron Power/1(Dynamic Pressure (Avoid Small Value))
  NOT/1 -> Switch/2
  Rollout Roll Control/1(Aileron Out) -> Saturation/1
  LPF AileronCmd/1(Output) -> Rollout Roll Control/2(Aileron In)
  Compare To Constant2/1 -> OR/1
  apMode/1 -> Compare To Constant2/1, Compare To Constant1/1, Rollout Roll Control/1(apMode)
  Compare To Constant1/1 -> OR/2
  OR1/1 -> Discrete-Time Integrator1/2, Unit Delay/1
  1/AileronPower/1 -> Gain/1, Sum1/2
  Roll Moment Caused By Damping/1(DAMP) -> 1/AileronPower/1
  Discrete-Time Integrator1/1 -> Sum3/1  "Sim_KI_roll"
  Kp_Roll/1 -> Sum3/2  "Sim_Kp_roll"
  Sum3/1 -> Switch/1
  Constant2/1 -> Discrete-Time Integrator1/3
  KI_Roll/1 -> Discrete-Time Integrator1/1
  Dimensional Aileron Power/1(CP) -> Divide/1
  Sum/1 -> Divide/2  "Sim.RollRate Error"
  Gain4/1 -> Switch/3  "Sim_Kp_roll"
  RollRate_Euler/1 -> Sum/2, K_TD/1
  RollRateCmd_Euler/1 -> 1-K_TD/1, Sum/1
  Unit Delay/1 -> NOT/1
  Switch/1 -> Gain1/1
  Gain1/1 -> Sum1/1
  Gain/1 -> Terminator/1  "Sim_RollDamping"
  Saturation/1 -> Aileron_Deg/1
  1-K_TD/1 -> Sum2/1
  Divide/1 -> Gain4/1, Kp_Roll/1, KI_Roll/1
  Sum2/1 -> Roll Moment Caused By Damping/1(RollRate_Body)  "RollDamp_TrustMix"
  V/1 -> Roll Moment Caused By Damping/2(V)
  "AileronTrim "/1 -> Sum1/4
  "1/AileronPower  "/1 -> Sum1/3
  K_TD/1 -> Sum2/2
  STIFF/1 -> "1/AileronPower  "/1
  Sum1/1 -> LPF AileronCmd/1("Input ")
  Q/1 -> Saturation1/1
  [ApGlobal] -> NOT1/1
  OR/1 -> OR1/1
  NOT1/1 -> Terminator1/1, OR1/2

== system Lib_Piccolo/Bank to Aileron/DynamicPLimit ==
  note: Q saturates at ~ 100mps which in IAS is 6125Pa
  apMode : Inport
  DynamicPressure_Pa : Inport  Port=2
  Compare To Constant1 : simulink/Logic and Bit Operations/Compare To Constant  relop=>=  const=5  OutDataTypeStr=uint8
  Compare To Constant2 : simulink/Logic and Bit Operations/Compare To Constant  relop=>=  const=11  OutDataTypeStr=uint8
  Compare To Constant3 : simulink/Logic and Bit Operations/Compare To Constant  relop=>=  const=10  OutDataTypeStr=uint8
  Latch : Subsystem
  Qmax : Constant  Value=6125
  Saturation Dynamic : simulink/Discontinuities/Saturation Dynamic  OutMin=[]  OutMax=[]  OutDataTypeStr=Inherit: Same as second input  OutDataType=fixdt(1, 16)  OutScaling=2^-10  DoSatur=off
  Switch : Switch  Criteria=u2 > Threshold
  Switch1 : Switch  Criteria=u2 > Threshold
  Out1 : Outport
  wires:
  Latch/1(Q_Latched) -> Switch1/2
  Switch1/1 -> Saturation Dynamic/3
  [Qmin_Bounce] -> Switch1/1
  Switch/1 -> Switch1/3
  Compare To Constant2/1 -> Latch/1(D)
  Compare To Constant1/1 -> Latch/2(Enable/!Rst)
  Qmax/1 -> Saturation Dynamic/1
  [Qmin_Flare] -> Switch/1
  [Qmin] -> Switch/3
  Compare To Constant3/1 -> Switch/2
  apMode/1 -> Compare To Constant3/1, Compare To Constant2/1, Compare To Constant1/1
  Saturation Dynamic/1 -> Out1/1
  DynamicPressure_Pa/1 -> Saturation Dynamic/2

== system Lib_Piccolo/Bank to Aileron/Reference Model ==
  BankCmd_Euler : Inport
  "Bank_Euler " : Inport  Port=2
  "BankMax_Euler " : Inport  Port=3
  Constant : Constant  Value=RollMaxAccel
  Fp_roll : Gain  Gain=Fp_Roll
  Gain1 : Gain  Gain=-1
  Gain2 : Gain  Gain=-1
  Gain3 : Gain  Gain=-1
  Gain4 : Gain  Gain=180/pi
  Gain9 : Gain  Gain=180/pi
  Roll Rate Max Accel Rate Limit : Subsystem
  "RollRateCmd " : Constant  Value=0
  "RollRateLimit_Max " : Constant  Value=RollRateMax
  Saturation Dynamic : simulink/Discontinuities/Saturation Dynamic  OutMin=[]  OutMax=[]  OutDataTypeStr=Inherit: Same as second input  OutDataType=fixdt(1, 16)  OutScaling=2^-10  DoSatur=off
  Saturation Dynamic1 : simulink/Discontinuities/Saturation Dynamic  OutMin=[]  OutMax=[]  OutDataTypeStr=Inherit: Same as second input  OutDataType=fixdt(1, 16)  OutScaling=2^-10  DoSatur=off
  Sum : Sum  Inputs=|+-
  Sum1 : Sum  Inputs=|++
  Terminator : Terminator
  Terminator2 : Terminator
  RollRateCmd_Euler : Outport
  tag scope: Sim_BankCmd=global
  wires:
  Saturation Dynamic1/1 -> Sum/1, Gain4/1, [Sim_BankCmd]
  Saturation Dynamic/1 -> RollRateCmd_Euler/1
  Gain9/1 -> Terminator2/1  "Sim.BankLimit"
  BankCmd_Euler/1 -> Saturation Dynamic1/2
  "RollRateLimit_Max "/1 -> Gain3/1, Saturation Dynamic/1
  Constant/1 -> Gain1/1, Roll Rate Max Accel Rate Limit/1(up)
  Fp_roll/1 -> Sum1/1
  Gain2/1 -> Saturation Dynamic1/3
  Gain4/1 -> Terminator/1  "Sim.BankCmd_Limit"
  Roll Rate Max Accel Rate Limit/1(Y) -> Saturation Dynamic/2
  Sum1/1 -> Roll Rate Max Accel Rate Limit/2(u)
  Gain3/1 -> Saturation Dynamic/3
  "BankMax_Euler "/1 -> Gain2/1, Saturation Dynamic1/1, Gain9/1
  Sum/1 -> Fp_roll/1
  "Bank_Euler "/1 -> Sum/2
  Gain1/1 -> Roll Rate Max Accel Rate Limit/3(lo)
  "RollRateCmd "/1 -> Sum1/2

== system Lib_Piccolo/Bank to Aileron/TASLimit ==
  note: TAS saturates at ~ 100mps which in IAS is 6125Pa
  apMode : Inport
  <V_mps> : Inport  Port=2
  Compare To Constant1 : simulink/Logic and Bit Operations/Compare To Constant  relop=>=  const=5  OutDataTypeStr=uint8
  Compare To Constant2 : simulink/Logic and Bit Operations/Compare To Constant  relop=>=  const=11  OutDataTypeStr=uint8
  Compare To Constant4 : simulink/Logic and Bit Operations/Compare To Constant  relop=>=  const=10  OutDataTypeStr=uint8
  Constant : Constant  Value=IASmin
  Constant1 : Constant  Value=IASstall
  Constant2 : Constant  Value=IASbounce
  Latch : Subsystem
  Saturation Dynamic1 : simulink/Discontinuities/Saturation Dynamic  OutMin=[]  OutMax=[]  OutDataTypeStr=Inherit: Same as second input  OutDataType=fixdt(1, 16)  OutScaling=2^-10  DoSatur=off
  Switch1 : Switch  Criteria=u2 > Threshold
  Switch2 : Switch  Criteria=u2 > Threshold
  TASmax : Constant  Value=100
  Out1 : Outport
  wires:
  TASmax/1 -> Saturation Dynamic1/1
  Constant2/1 -> Switch2/1
  Compare To Constant1/1 -> Latch/2(Enable/!Rst)
  Switch1/1 -> Switch2/3
  apMode/1 -> Compare To Constant4/1, Compare To Constant2/1, Compare To Constant1/1
  Compare To Constant2/1 -> Latch/1(D)
  Latch/1(Q_Latched) -> Switch2/2
  <V_mps>/1 -> Saturation Dynamic1/2
  Constant/1 -> Switch1/3
  Saturation Dynamic1/1 -> Out1/1
  Constant1/1 -> Switch1/1
  Compare To Constant4/1 -> Switch1/2
  Switch2/1 -> Saturation Dynamic1/3

== system Lib_Piccolo/Brake Controller/Variant Subsystem ==
  note: 1) Add Subsystem or Model blocks as valid variant choices.
      | 2) You cannot connect blocks at this level. At simulation, connectivity is automatically
      | determined, based on the active variant and port name matching.
  Feedback Bus : Inport
  16P : Subsystem  VariantControl="modelScale ==\"16P5\""
  7P : Subsystem  VariantControl="modelScale == \"7P\""
  Brake_Pcnt : Outport
